simulink model "chenRinconMoraModel"  (R2021b)
settings: Solver=FixedStepAuto  StartTime=0.0  StopTime=T  FixedStep=dt  RelTol=1e-3  AbsTol=1e-3
values from neighbouring files (symbols this model uses):
  fn = '20230919_batteryTest.txt'    [20230919_data_fit.mat]    (also in CBM_testscript_importdata.m = 'data/data_test1'; chenRinconMoraModel_optimization.m = 'data/data_test1.mat'; chenRinconMoraModel_simulate.m = 'data/data_test1.mat'; chenRinconMoraModel_simulate_expdata.m = 'data_cut\data_20220810.mat')
  p = zeros(size(yp,1),3)    [crm_paramfit.m]    (also in psObj_correction.m = Pulse(i))
libraries: fl_lib x13, nesl_utility x11, ee_lib x2
settings Model: Creator=drkfr  LastModifiedBy=drkfr
settings SolverCC: AutoScaleAbsTol=off
settings DebuggingCC: SymbolicDimsDataTypeCodeGenerationDiagnostic=none  SFMachineParentedDataDiag=warning
settings SFSimCC: CustomCodeUndefinedFunction=UseInterfaceOnly
settings SimscapeCC: SimscapeLogType=all  SimscapeLogSimulationStatistics=on  SimscapeLogDataHistory=10000

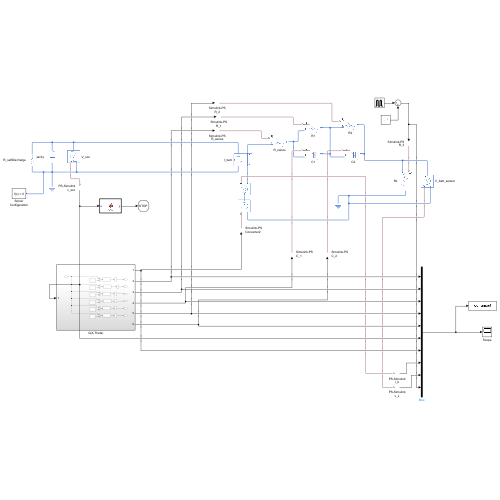
[thumbnail: Simulink's stored preview of the top-level diagram]
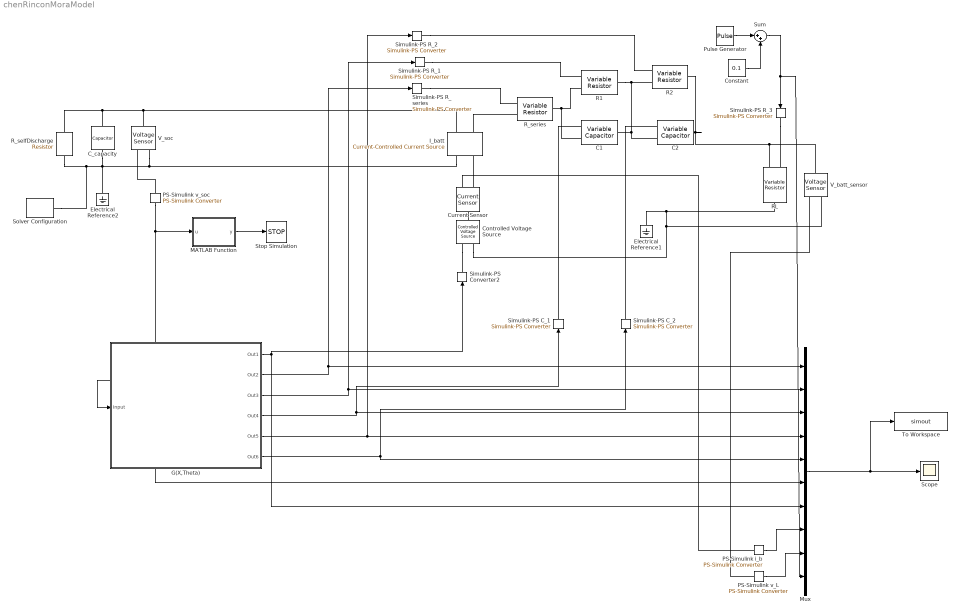
== system chenRinconMoraModel ==
  C1 : ee_lib/Passive/Variable Capacitor  prm=2  Cmin=1e-9 F  r=1e-6 Ohm  v0=0 V  q0=0 C
      settings: SourceProductBaseCode=PS  InternalSimscapePortConfiguration="{\"Bottom\":[],\"Left\":[{\"id\":\"C\",\"label\":\"C\",\"type\":\"input\"},{\"id\":\"p\",\"label\":\"+\",\"type\":\"foundation.electrical.electrical\"}],\"Right\":[{\"id\":\"n\",\"label\":\"-\",\"type\":\"foundation.electrical.electrical\"}],\"Top\":[]}"
  C2 : ee_lib/Passive/Variable Capacitor  prm=2  Cmin=1e-9 F  r=1e-6 Ohm  v0=0 V  q0=0 C
      settings: SourceProductBaseCode=PS  InternalSimscapePortConfiguration="{\"Bottom\":[],\"Left\":[{\"id\":\"C\",\"label\":\"C\",\"type\":\"input\"},{\"id\":\"p\",\"label\":\"+\",\"type\":\"foundation.electrical.electrical\"}],\"Right\":[{\"id\":\"n\",\"label\":\"-\",\"type\":\"foundation.electrical.electrical\"}],\"Top\":[]}"
  C_capacity : fl_lib/Electrical/Electrical Elements/Capacitor  c=p.C_capacity F  r=1e-6 Ohm  g=0 1/Ohm  i_specify=off  i_priority=None  i=0 A  i_nominal_specify=off  i_nominal_unit=A  i_nominal_value=1  v_specify=off  v_priority=None  v=50 V  v_nominal_specify=off  v_nominal_unit=V  v_nominal_value=1  vc_specify=on  vc_priority=High  vc=1 V  vc_nominal_specify=off  vc_nominal_unit=V  vc_nominal_value=1
  Constant : Constant  Value=0.1
  Controlled Voltage Source : fl_lib/Electrical/Electrical Sources/Controlled Voltage Source
  Current Sensor : fl_lib/Electrical/Electrical Sensors/Current Sensor
  Electrical Reference1 : fl_lib/Electrical/Electrical Elements/Electrical Reference
  Electrical Reference2 : fl_lib/Electrical/Electrical Elements/Electrical Reference
  G(X,Theta) : Subsystem
  I_batt : fl_lib/Electrical/Electrical Sources/Current-Controlled Current Source  K=1  i1_specify=off  i1_priority=None  i1=0 A  i1_nominal_specify=off  i1_nominal_unit=A  i1_nominal_value=1  i2_specify=off  i2_priority=None  i2=0 A  i2_nominal_specify=off  i2_nominal_unit=A  i2_nominal_value=1
      settings: SourceProductBaseCode=SS  InternalSimscapePortConfiguration="{\"Bottom\":[],\"Left\":[{\"id\":\"p1\",\"label\":\"+\",\"type\":\"foundation.electrical.electrical\"},{\"id\":\"head\",\"label\":\"\",\"type\":\"foundation.electrical.electrical\"}],\"Right\":[{\"id\":\"n1\",\"label\":\"-\",\"type\":\"foundation.electrical.electrical\"},{\"id\":\"tail\",\"label\":\"\",\"type\":\"foundation.electrical.electrical\"}],\"Top\":[]}"
  MATLAB Function : MATLAB Function  TreatAsAtomicUnit=on
  Mux : Mux  Inputs=10
  PS-Simulink i_b : nesl_utility/PS-Simulink Converter  PhysicalDomain=network_engine_domain  SubClassName=ps_output  LeftPortType=input  RightPortType=output  PseudoPeriodic=off  Frequencies=[]  Unit=A  AffineConversion=off
      settings: SourceProductBaseCode=PW,SS
  PS-Simulink v_L : nesl_utility/PS-Simulink Converter  PhysicalDomain=network_engine_domain  SubClassName=ps_output  LeftPortType=input  RightPortType=output  PseudoPeriodic=off  Frequencies=[]  Unit=V  AffineConversion=off
      settings: SourceProductBaseCode=PW,SS
  PS-Simulink v_soc : nesl_utility/PS-Simulink Converter  PhysicalDomain=network_engine_domain  SubClassName=ps_output  LeftPortType=input  RightPortType=output  PseudoPeriodic=off  Frequencies=[]  Unit=V  AffineConversion=off
      settings: SourceProductBaseCode=PW,SS
  Pulse Generator : DiscretePulseGenerator  PulseType=Time based  Amplitude=1e6  Period=120  PulseWidth=10
  R1 : fl_lib/Electrical/Electrical Elements/Variable Resistor  Rmin=0 Ohm  i_specify=off  i_priority=None  i=0 A  i_nominal_specify=off  i_nominal_unit=A  i_nominal_value=1  v_specify=off  v_priority=None  v=0 V  v_nominal_specify=off  v_nominal_unit=V  v_nominal_value=1
  R2 : fl_lib/Electrical/Electrical Elements/Variable Resistor  Rmin=0 Ohm  i_specify=off  i_priority=None  i=0 A  i_nominal_specify=off  i_nominal_unit=A  i_nominal_value=1  v_specify=off  v_priority=None  v=0 V  v_nominal_specify=off  v_nominal_unit=V  v_nominal_value=1
  RL : fl_lib/Electrical/Electrical Elements/Variable Resistor  Rmin=0.001 Ohm  i_specify=off  i_priority=None  i=0 A  i_nominal_specify=off  i_nominal_unit=A  i_nominal_value=1  v_specify=off  v_priority=None  v=0 V  v_nominal_specify=off  v_nominal_unit=V  v_nominal_value=1
  R_selfDischarge : fl_lib/Electrical/Electrical Elements/Resistor  R=p.R_selfDischarge Ohm  i_specify=off  i_priority=None  i=0 A  i_nominal_specify=off  i_nominal_unit=A  i_nominal_value=1  v_specify=off  v_priority=None  v=0 V  v_nominal_specify=off  v_nominal_unit=V  v_nominal_value=1
  R_series : fl_lib/Electrical/Electrical Elements/Variable Resistor  Rmin=0 Ohm  i_specify=off  i_priority=None  i=0 A  i_nominal_specify=off  i_nominal_unit=A  i_nominal_value=1  v_specify=off  v_priority=None  v=0 V  v_nominal_specify=off  v_nominal_unit=V  v_nominal_value=1
  Scope : Scope
  Simulink-PS C_1 : nesl_utility/Simulink-PS Converter  PhysicalDomain=network_engine_domain  SubClassName=ps_input  LeftPortType=input  RightPortType=output  PseudoPeriodic=off  Frequencies=[]  NoiseDistribution=none  NoiseParameters=[]  Unit=F  AffineConversion=off  FilteringAndDerivatives=provide  SimscapeFilterOrder=1  InputFilterTimeConstant=0.001  UdotUserProvided=0
      settings: SourceProductBaseCode=PW,SS
  Simulink-PS C_2 : nesl_utility/Simulink-PS Converter  PhysicalDomain=network_engine_domain  SubClassName=ps_input  LeftPortType=input  RightPortType=output  PseudoPeriodic=off  Frequencies=[]  NoiseDistribution=none  NoiseParameters=[]  Unit=F  AffineConversion=off  FilteringAndDerivatives=provide  SimscapeFilterOrder=1  InputFilterTimeConstant=0.001  UdotUserProvided=0
      settings: SourceProductBaseCode=PW,SS
  Simulink-PS Converter2 : nesl_utility/Simulink-PS Converter  PhysicalDomain=network_engine_domain  SubClassName=ps_input  LeftPortType=input  RightPortType=output  PseudoPeriodic=off  Frequencies=[]  NoiseDistribution=none  NoiseParameters=[]  Unit=V  AffineConversion=off  FilteringAndDerivatives=provide  SimscapeFilterOrder=1  InputFilterTimeConstant=0.001  UdotUserProvided=0
      settings: SourceProductBaseCode=PW,SS
  Simulink-PS R_1 : nesl_utility/Simulink-PS Converter  PhysicalDomain=network_engine_domain  SubClassName=ps_input  LeftPortType=input  RightPortType=output  PseudoPeriodic=off  Frequencies=[]  NoiseDistribution=none  NoiseParameters=[]  Unit=Ohm  AffineConversion=off  FilteringAndDerivatives=provide  SimscapeFilterOrder=1  InputFilterTimeConstant=0.001  UdotUserProvided=0
      settings: SourceProductBaseCode=PW,SS
  Simulink-PS R_2 : nesl_utility/Simulink-PS Converter  PhysicalDomain=network_engine_domain  SubClassName=ps_input  LeftPortType=input  RightPortType=output  PseudoPeriodic=off  Frequencies=[]  NoiseDistribution=none  NoiseParameters=[]  Unit=Ohm  AffineConversion=off  FilteringAndDerivatives=provide  SimscapeFilterOrder=1  InputFilterTimeConstant=0.001  UdotUserProvided=0
      settings: SourceProductBaseCode=PW,SS
  Simulink-PS R_3 : nesl_utility/Simulink-PS Converter  PhysicalDomain=network_engine_domain  SubClassName=ps_input  LeftPortType=input  RightPortType=output  PseudoPeriodic=off  Frequencies=[]  NoiseDistribution=none  NoiseParameters=[]  Unit=Ohm  AffineConversion=off  FilteringAndDerivatives=provide  SimscapeFilterOrder=1  InputFilterTimeConstant=0.001  UdotUserProvided=0
      settings: SourceProductBaseCode=PW,SS
  Simulink-PS R_series : nesl_utility/Simulink-PS Converter  PhysicalDomain=network_engine_domain  SubClassName=ps_input  LeftPortType=input  RightPortType=output  PseudoPeriodic=off  Frequencies=[]  NoiseDistribution=none  NoiseParameters=[]  Unit=Ohm  AffineConversion=off  FilteringAndDerivatives=provide  SimscapeFilterOrder=1  InputFilterTimeConstant=0.001  UdotUserProvided=0
      settings: SourceProductBaseCode=PW,SS
  Solver Configuration : nesl_utility/Solver Configuration  PhysicalDomain=network_engine_domain  SubClassName=solver  LeftPortType=input  RightPortType=generic  Tones=[]  Harmonics=[]  SimulateNoise=off  Profile=off  UseLocalSampling=off  EnableSwitchedLinearOptims=on  FrequencyDomain=off  UseCCode=off  RelTol=0.001  AbsTol=1e-06  MinStep=1e-09  ToWorkspace=off  RevertToSquareIcSolve=off  NumHomotopyIterations=100  PhasorMode=off  PhasorModeNumHarmonics=1  DoDC=on  ResidualTolerance=1e-09  UseLocalSolver=off  LocalSolverChoice=NE_BACKWARD_EULER_ADVANCER  LocalSolverSampleTime=0.001  DoFixedCost=off  MaxNonlinIter=3  MaxModeIter=2  ComputeImpulses=off  ImpulseIterations=2  LinearAlgebra=auto  EquationFormulation=NE_TIME_EF  DelaysMemoryBudget=1024  AutomaticFiltering=on  FilteringTimeConstant=0.001  PartitionStorageMethod=AS_NEEDED  PartitionMemoryBudget=1024  PartitionMethod=ROBUST
      settings: SourceProductBaseCode=PW,SS
  Stop Simulation : Stop
  Sum : Sum  Inputs=|++
  To Workspace : ToWorkspace  VariableName=simout  SaveFormat=Timeseries  SampleTime=-1
  V_batt_sensor : fl_lib/Electrical/Electrical Sensors/Voltage Sensor
  V_soc : fl_lib/Electrical/Electrical Sensors/Voltage Sensor
  wires:
  PS-Simulink v_soc/1 -> MATLAB Function/1(u), Mux/6, G(X,Theta)/1(Input)
  G(X,Theta)/1(Out1) -> Simulink-PS Converter2/1, Mux/7
  G(X,Theta)/2(Out2) -> Simulink-PS R_series/1, Mux/1
  G(X,Theta)/3(Out3) -> Simulink-PS R_1/1, Mux/2
  G(X,Theta)/4(Out4) -> Simulink-PS C_1/1, Mux/3
  G(X,Theta)/5(Out5) -> Simulink-PS R_2/1, Mux/4
  G(X,Theta)/6(Out6) -> Simulink-PS C_2/1, Mux/5
  Pulse Generator/1 -> Sum/1
  Constant/1 -> Sum/2
  Sum/1 -> Mux/10, Simulink-PS R_3/1
  Mux/1 -> To Workspace/1, Scope/1
  PS-Simulink i_b/1 -> Mux/8
  PS-Simulink v_L/1 -> Mux/9
  MATLAB Function/1(y) -> Stop Simulation/1
  connections:
  R_series/RConn1 -- C1/LConn2 -- R1/LConn2
  R1/RConn1 -- R2/LConn2 -- C1/RConn1 -- C2/LConn2
  V_batt_sensor/LConn1 -- R2/RConn1 -- C2/RConn1 -- RL/LConn2
  I_batt/LConn2 -- R_selfDischarge/RConn1 -- Solver Configuration/RConn1 -- C_capacity/RConn1 -- Electrical Reference2/LConn1 -- V_soc/RConn2
  C_capacity/LConn1 -- V_soc/LConn1 -- I_batt/RConn2 -- R_selfDischarge/LConn1
  Controlled Voltage Source/RConn2 -- RL/RConn1 -- Electrical Reference1/LConn1 -- V_batt_sensor/RConn2
  R_series/LConn2 -- I_batt/RConn1
  Current Sensor/LConn1 -- Controlled Voltage Source/LConn1
  Current Sensor/RConn2 -- I_batt/LConn1
  Controlled Voltage Source/RConn1 -- Simulink-PS Converter2/RConn1
  PS-Simulink v_soc/LConn1 -- V_soc/RConn1
  Simulink-PS R_series/RConn1 -- R_series/LConn1
  Simulink-PS R_1/RConn1 -- R1/LConn1
  Simulink-PS C_1/RConn1 -- C1/LConn1
  Simulink-PS R_2/RConn1 -- R2/LConn1
  Simulink-PS C_2/RConn1 -- C2/LConn1
  Simulink-PS R_3/RConn1 -- RL/LConn1
  PS-Simulink i_b/LConn1 -- Current Sensor/RConn1
  PS-Simulink v_L/LConn1 -- V_batt_sensor/RConn1

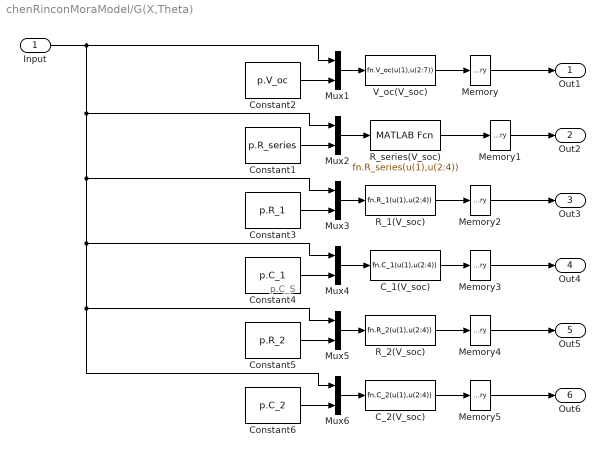
== system chenRinconMoraModel/G(X,Theta) ==
  note: p.C_S
  Input : Inport
  C_1(V_soc) : MATLABFcn  MATLABFcn=fn.C_1(u(1),u(2:4))  OutputDimensions=1  OutputSignalType=real
  C_2(V_soc) : MATLABFcn  MATLABFcn=fn.C_2(u(1),u(2:4))  OutputDimensions=1  OutputSignalType=real
  Constant1 : Constant  Value=p.R_series
  Constant2 : Constant  Value=p.V_oc
  Constant3 : Constant  Value=p.R_1
  Constant4 : Constant  Value=p.C_1
  Constant5 : Constant  Value=p.R_2
  Constant6 : Constant  Value=p.C_2
  Memory{,1..5} (6 alike) : Memory
  Mux{1..6} (6 alike) : Mux  Inputs=2
  R_1(V_soc) : MATLABFcn  MATLABFcn=fn.R_1(u(1),u(2:4))  OutputDimensions=1  OutputSignalType=real
  R_2(V_soc) : MATLABFcn  MATLABFcn=fn.R_2(u(1),u(2:4))  OutputDimensions=1  OutputSignalType=real
  R_series(V_soc) : MATLABFcn  MATLABFcn=fn.R_series(u(1),u(2:4))  OutputDimensions=1  OutputSignalType=real
  V_oc(V_soc) : MATLABFcn  MATLABFcn=fn.V_oc(u(1),u(2:7))  OutputDimensions=1  OutputSignalType=real
  Out1 : Outport
  Out2 : Outport  Port=2
  Out3 : Outport  Port=3
  Out4 : Outport  Port=4
  Out5 : Outport  Port=5
  Out6 : Outport  Port=6
  wires:
  V_oc(V_soc)/1 -> Memory/1
  Constant2/1 -> Mux1/2
  Mux1/1 -> V_oc(V_soc)/1
  Memory/1 -> Out1/1
  Memory1/1 -> Out2/1
  Mux2/1 -> R_series(V_soc)/1
  R_series(V_soc)/1 -> Memory1/1
  Constant1/1 -> Mux2/2
  Memory2/1 -> Out3/1
  Mux3/1 -> R_1(V_soc)/1
  R_1(V_soc)/1 -> Memory2/1
  Constant3/1 -> Mux3/2
  Memory3/1 -> Out4/1
  Mux4/1 -> C_1(V_soc)/1
  C_1(V_soc)/1 -> Memory3/1
  Constant4/1 -> Mux4/2
  Constant6/1 -> Mux6/2
  C_2(V_soc)/1 -> Memory5/1
  Input/1 -> Mux6/1, Mux5/1, Mux4/1, Mux3/1, Mux2/1, Mux1/1
  Memory5/1 -> Out6/1
  Mux6/1 -> C_2(V_soc)/1
  R_2(V_soc)/1 -> Memory4/1
  Constant5/1 -> Mux5/2
  Memory4/1 -> Out5/1
  Mux5/1 -> R_2(V_soc)/1

== matlab function chenRinconMoraModel/MATLAB Function ==
  data: u input; y output
function y = fcn(u)
if u <= 0
    y = 1;
else
    y = 0;
end
